simulink model "brazo_planta"  (R2026b)
settings: Solver=VariableStepAuto  StopTime=15
undefined symbols (not defined in the file or in its folder): X, Y, Z
libraries: sm_lib x97, nesl_utility x16, instrumentseriallib x3
(part 3 of 3)

== matlab function brazo_planta/MATLAB Function1 ==
  data: theta input; q_ref output
function q_ref = logico_a_simscape(theta)
theta = reshape(theta, 1, []);   % siempre fila, venga de donde venga
% Convierte los ángulos LÓGICOS del ESP32 a las articulaciones de Simscape.
%   theta : [B S E W H G] en grados (convención -90..90 del código)
%   q_ref : 7 articulaciones en rad, orden de showdetails:
%           base, hombro, codo, muneca_pitch, muneca_roll, pinza, pinza_2
%
% Guardar este archivo en la carpeta del modelo; el bloque MATLAB Function
% solo tiene que llamar:  q_ref = logico_a_simscape(theta);

% --- Qué servo mueve cada articulación de Simscape (VERIFICAR) ---
% En el ESP32 el canal W recibe el roll y el canal H recibe el pitch,
% por eso muneca_pitch <- H (5) y muneca_roll <- W (4).
% Si en tu robot es al revés, cambia a [1 2 3 4 5 6 6].
FUENTE = [1 2 3 4 5 6 6];

% --- Calibración (AJUSTAR con calibrar_mapeo.m) ---
SIGNO    = [-1 -1 -1 1 -1 -1 1];   % -1 si la articulación gira al revés; pinza_2 en espejo
OFFSET   = [0 -17 -53 0 -36 -20 -20];   % ángulo lógico [°] que corresponde a q = 0 en Simscape
RELACION = [1 1 1 1 1 1 1];   % ángulo articulación / ángulo servo (engranajes, etc.)

q_ref = SIGNO .* RELACION .* (theta(FUENTE) - OFFSET) * pi/180;
end
